simulink model "rfsoc4x2_ospfb_128"  (R2021a)
(part 12 of 339)

  pol1_in1_tap11/2(sync_out) -> pol1_in1_tap12/2(sync)
  pol1_in1_tap11/1(dout) -> pol1_in1_tap12/1(din)
  pol1_in1_first_tap5/6(pot_en_out) -> pol1_in1_tap11/5(pot_en_in)
  [addr] -> pol1_in1_first_tap5/4(addr_in)
  pol1_in1_tap12/4(taps_out) -> delay32/1
  delay29/1 -> adder_1_6/1(sync)
  delay26/1 -> adder_1_5/2(din1)
  pol1_in1_last_tap4/1(tap_out) -> adder_1_5/5(din4)
  pol1_in1_first_tap4/1(dout) -> pol1_in1_tap9/1(din)
  pol1_in2_coeffs3/2(sync_out) -> pol1_in1_first_tap4/2(sync)
  pol1_in1_tap9/3(coeff_out) -> pol1_in1_tap10/3(coeff)
  pol1_in1_first_tap4/2(sync_out) -> pol1_in1_tap9/2(sync)
  pol1_in1_tap10/1(dout) -> pol1_in1_last_tap4/1(din)
  pol1_in1_tap9/5(add_out) -> pol1_in1_tap10/4(addr_in)
  pol1_in1_tap9/6(pot_en_out) -> pol1_in1_tap10/5(pot_en_in)
  pol1_in1_tap10/2(sync_out) -> pol1_in1_last_tap4/2(sync)
  pol1_in1_tap10/3(coeff_out) -> pol1_in1_last_tap4/3(coeff)
  pol1_in2_coeffs3/3(coeff) -> pol1_in1_first_tap4/3(coeffs)
  pol1_in1_last_tap4/2(sync_out) -> delay25/1
  pol1_in1_first_tap4/3(coeff_out) -> pol1_in1_tap9/3(coeff)
  delay27/1 -> adder_1_5/3(din2)
  [tap_write_en] -> pol1_in1_first_tap4/5(pot_en_in)
  pol1_in2_coeffs3/1(dout) -> pol1_in1_first_tap4/1(din)
  delay28/1 -> adder_1_5/4(din3)
  pol1_in1_tap9/4(taps_out) -> delay27/1
  pol1_in1_first_tap4/4(taps_out) -> delay26/1
  pol1_in1_first_tap4/5(add_out) -> pol1_in1_tap9/4(addr_in)
  pol1_in1_tap9/2(sync_out) -> pol1_in1_tap10/2(sync)
  pol1_in1_tap9/1(dout) -> pol1_in1_tap10/1(din)
  pol1_in1_first_tap4/6(pot_en_out) -> pol1_in1_tap9/5(pot_en_in)
  [addr] -> pol1_in1_first_tap4/4(addr_in)
  pol1_in1_tap10/4(taps_out) -> delay28/1
  delay25/1 -> adder_1_5/1(sync)
  delay22/1 -> adder_1_4/2(din1)
  pol1_in1_last_tap3/1(tap_out) -> adder_1_4/5(din4)
  pol1_in1_first_tap3/1(dout) -> pol1_in1_tap7/1(din)
  pol1_in2_coeffs2/2(sync_out) -> pol1_in1_first_tap3/2(sync)
  pol1_in1_tap7/3(coeff_out) -> pol1_in1_tap8/3(coeff)
  pol1_in1_first_tap3/2(sync_out) -> pol1_in1_tap7/2(sync)
  pol1_in1_tap8/1(dout) -> pol1_in1_last_tap3/1(din)
  pol1_in1_tap7/5(add_out) -> pol1_in1_tap8/4(addr_in)
  pol1_in1_tap7/6(pot_en_out) -> pol1_in1_tap8/5(pot_en_in)
  pol1_in1_tap8/2(sync_out) -> pol1_in1_last_tap3/2(sync)
  pol1_in1_tap8/3(coeff_out) -> pol1_in1_last_tap3/3(coeff)
  pol1_in2_coeffs2/3(coeff) -> pol1_in1_first_tap3/3(coeffs)
  pol1_in1_last_tap3/2(sync_out) -> delay21/1
  pol1_in1_first_tap3/3(coeff_out) -> pol1_in1_tap7/3(coeff)
  delay23/1 -> adder_1_4/3(din2)
  [tap_write_en] -> pol1_in1_first_tap3/5(pot_en_in)
  pol1_in2_coeffs2/1(dout) -> pol1_in1_first_tap3/1(din)
  delay24/1 -> adder_1_4/4(din3)
  pol1_in1_tap7/4(taps_out) -> delay23/1
  pol1_in1_first_tap3/4(taps_out) -> delay22/1
  pol1_in1_first_tap3/5(add_out) -> pol1_in1_tap7/4(addr_in)
  pol1_in1_tap7/2(sync_out) -> pol1_in1_tap8/2(sync)
  pol1_in1_tap7/1(dout) -> pol1_in1_tap8/1(din)
  pol1_in1_first_tap3/6(pot_en_out) -> pol1_in1_tap7/5(pot_en_in)
  [addr] -> pol1_in1_first_tap3/4(addr_in)
  pol1_in1_tap8/4(taps_out) -> delay24/1
  delay21/1 -> adder_1_4/1(sync)
  delay18/1 -> adder_1_3/2(din1)
  pol1_in1_last_tap2/1(tap_out) -> adder_1_3/5(din4)
  pol1_in1_first_tap2/1(dout) -> pol1_in1_tap5/1(din)
  pol1_in2_coeffs1/2(sync_out) -> pol1_in1_first_tap2/2(sync)
  pol1_in1_tap5/3(coeff_out) -> pol1_in1_tap6/3(coeff)
  pol1_in1_first_tap2/2(sync_out) -> pol1_in1_tap5/2(sync)
  pol1_in1_tap6/1(dout) -> pol1_in1_last_tap2/1(din)
  pol1_in1_tap5/5(add_out) -> pol1_in1_tap6/4(addr_in)
  pol1_in1_tap5/6(pot_en_out) -> pol1_in1_tap6/5(pot_en_in)
  pol1_in1_tap6/2(sync_out) -> pol1_in1_last_tap2/2(sync)
  pol1_in1_tap6/3(coeff_out) -> pol1_in1_last_tap2/3(coeff)
  pol1_in2_coeffs1/3(coeff) -> pol1_in1_first_tap2/3(coeffs)
  pol1_in1_last_tap2/2(sync_out) -> delay17/1
  pol1_in1_first_tap2/3(coeff_out) -> pol1_in1_tap5/3(coeff)
  delay19/1 -> adder_1_3/3(din2)
  [tap_write_en] -> pol1_in1_first_tap2/5(pot_en_in)
  pol1_in2_coeffs1/1(dout) -> pol1_in1_first_tap2/1(din)
  delay20/1 -> adder_1_3/4(din3)
  pol1_in1_tap5/4(taps_out) -> delay19/1
  pol1_in1_first_tap2/4(taps_out) -> delay18/1
  pol1_in1_first_tap2/5(add_out) -> pol1_in1_tap5/4(addr_in)
  pol1_in1_tap5/2(sync_out) -> pol1_in1_tap6/2(sync)
  pol1_in1_tap5/1(dout) -> pol1_in1_tap6/1(din)
  pol1_in1_first_tap2/6(pot_en_out) -> pol1_in1_tap5/5(pot_en_in)
  [addr] -> pol1_in1_first_tap2/4(addr_in)
  pol1_in1_tap6/4(taps_out) -> delay20/1
  delay17/1 -> adder_1_3/1(sync)
  pol1_in1_last_tap1/1(tap_out) -> adder_1_2/5(din4)
  delay10/1 -> adder_1_2/1(sync)
  [tap_write_en] -> pol1_in1_first_tap1/5(pot_en_in)
  pol1_in1_tap4/4(taps_out) -> delay13/1
  pol1_in1_first_tap1/1(dout) -> pol1_in1_tap1/1(din)
  pol1_in1_tap1/4(taps_out) -> delay12/1
  pol1_in2_coeffs/1(dout) -> pol1_in1_first_tap1/1(din)
  pol1_in1_first_tap1/2(sync_out) -> pol1_in1_tap1/2(sync)
  delay13/1 -> adder_1_2/4(din3)
  pol1_in1_tap1/2(sync_out) -> pol1_in1_tap4/2(sync)
  pol1_in1_tap1/3(coeff_out) -> pol1_in1_tap4/3(coeff)
  pol1_in1_tap4/2(sync_out) -> pol1_in1_last_tap1/2(sync)
  pol1_in2_coeffs/3(coeff) -> pol1_in1_first_tap1/3(coeffs)
  pol1_in1_tap4/1(dout) -> pol1_in1_last_tap1/1(din)
  pol1_in1_first_tap1/5(add_out) -> pol1_in1_tap1/4(addr_in)
  pol1_in1_tap1/5(add_out) -> pol1_in1_tap4/4(addr_in)
  pol1_in1_tap1/1(dout) -> pol1_in1_tap4/1(din)
  pol1_in1_tap1/6(pot_en_out) -> pol1_in1_tap4/5(pot_en_in)
  delay12/1 -> adder_1_2/3(din2)
  pol1_in1_first_tap1/6(pot_en_out) -> pol1_in1_tap1/5(pot_en_in)
  pol1_in1_first_tap1/4(taps_out) -> delay11/1
  pol1_in2_coeffs/2(sync_out) -> pol1_in1_first_tap1/2(sync)
  pol1_in1_tap4/3(coeff_out) -> pol1_in1_last_tap1/3(coeff)
  delay11/1 -> adder_1_2/2(din1)
  pol1_in1_first_tap1/3(coeff_out) -> pol1_in1_tap1/3(coeff)
  [addr] -> pol1_in1_first_tap1/4(addr_in)
  pol1_in1_last_tap1/2(sync_out) -> delay10/1
  Gateway Out6/1 -> scope4/3
  Gateway Out5/1 -> scope4/2
  Gateway Out4/1 -> scope4/4
  Gateway Out7/1 -> scope4/1
  delay7/1 -> Gateway Out7/1, adder_1_1/2(din1)
  delay8/1 -> Gateway Out5/1, adder_1_1/3(din2)
  delay9/1 -> adder_1_1/4(din3), Gateway Out6/1
  Gateway Out3/1 -> scope3/1
  Gateway Out2/1 -> scope2/1
  delay6/1 -> Gateway Out1/1, adder_1_1/1(sync)
  pol1_in1_last_tap/2(sync_out) -> delay6/1
  Gateway Out1/1 -> scope1/1
  delay5/1 -> Gateway Out266/1
  delay4/1 -> Gateway Out265/1
  delay3/1 -> Gateway Out267/1
  pol1_in1_coeffs/1(dout) -> pol1_in1_first_tap/1(din), delay3/1
  Gateway Out267/1 -> scope93/1
  Gateway Out264/1 -> scope93/4
  Gateway Out265/1 -> scope93/2
  Gateway Out266/1 -> scope93/3
  pol1_in1_tap2/6(pot_en_out) -> pol1_in1_tap3/5(pot_en_in)
  pol1_in1_tap2/5(add_out) -> pol1_in1_tap3/4(addr_in)
  pol1_in1_first_tap/6(pot_en_out) -> pol1_in1_tap2/5(pot_en_in)
  pol1_in1_first_tap/5(add_out) -> pol1_in1_tap2/4(addr_in)
  [tap_write_en] -> pol1_in1_first_tap/5(pot_en_in)
  [addr] -> pol1_in1_first_tap/4(addr_in)
  delay2/1 -> Counter38/1, Counter36/1
  Counter38/1 -> Delay26/1, Slice20/1
  Constant61/1 -> Relational11/2
  Slice20/1 -> edge_detect8/1(in)
  Constant63/1 -> Relational12/2
  Gateway Out251/1 -> scope86/1
  edge_detect8/1(out) -> Logical11/2
  Logical11/1 -> Counter36/2
  Gateway Out250/1 -> scope89/1
  AddSub11/1 -> Gateway Out250/1, Relational11/1, Mux3/2, AddSub12/1
  Inverter/1 -> Gateway Out255/1, [tap_write_en]
  Gateway Out252/1 -> scope88/1
  AddSub12/1 -> Mux3/3
  Gateway Out255/1 -> scope90/1
  Mux3/1 -> Gateway Out251/1, [addr]
  Delay27/1 -> Logical11/1
  Relational12/1 -> Inverter/1
  Counter36/1 -> Gateway Out253/1, AddSub11/2
  Constant62/1 -> AddSub12/2
  Gateway Out253/1 -> scope85/1
  Relational11/1 -> Mux3/1
  Delay26/1 -> Gateway Out252/1, AddSub11/1, Relational12/1
  en_ctrl/1 -> Delay27/1
  pol1_in1_tap3/4(taps_out) -> delay9/1
  pol1_in1_tap3/3(coeff_out) -> pol1_in1_last_tap/3(coeff)
  pol1_in1_tap3/2(sync_out) -> pol1_in1_last_tap/2(sync)
  pol1_in1_tap3/1(dout) -> Gateway Out264/1, pol1_in1_last_tap/1(din)
  pol1_in1_last_tap/1(tap_out) -> adder_1_1/5(din4), Gateway Out4/1
  pol1_in1_tap2/4(taps_out) -> delay8/1
  pol1_in1_tap2/3(coeff_out) -> pol1_in1_tap3/3(coeff)
  pol1_in1_tap2/2(sync_out) -> pol1_in1_tap3/2(sync)
  pol1_in1_tap2/1(dout) -> pol1_in1_tap3/1(din), delay5/1
  pol1_in1_first_tap/4(taps_out) -> delay7/1
  pol1_in1_first_tap/3(coeff_out) -> pol1_in1_tap2/3(coeff)
  pol1_in1_first_tap/2(sync_out) -> pol1_in1_tap2/2(sync)
  pol1_in1_first_tap/1(dout) -> pol1_in1_tap2/1(din), delay4/1
  convert_1_16/1 -> pol1_out16/1
  scale_1_16/1 -> convert_1_16/1
  adder_1_16/2(dout) -> scale_1_16/1
  convert_1_15/1 -> pol1_out15/1
  scale_1_15/1 -> convert_1_15/1
  adder_1_15/2(dout) -> scale_1_15/1
  convert_1_14/1 -> pol1_out14/1
  scale_1_14/1 -> convert_1_14/1
  adder_1_14/2(dout) -> scale_1_14/1
  convert_1_13/1 -> pol1_out13/1
  scale_1_13/1 -> convert_1_13/1
  adder_1_13/2(dout) -> scale_1_13/1
  convert_1_12/1 -> pol1_out12/1
  scale_1_12/1 -> convert_1_12/1
  adder_1_12/2(dout) -> scale_1_12/1
  convert_1_11/1 -> pol1_out11/1
  scale_1_11/1 -> convert_1_11/1
  adder_1_11/2(dout) -> scale_1_11/1
  convert_1_10/1 -> pol1_out10/1
  scale_1_10/1 -> convert_1_10/1
  adder_1_10/2(dout) -> scale_1_10/1
  convert_1_9/1 -> pol1_out9/1
  scale_1_9/1 -> convert_1_9/1
  adder_1_9/2(dout) -> scale_1_9/1
  convert_1_8/1 -> pol1_out8/1
  scale_1_8/1 -> convert_1_8/1
  adder_1_8/2(dout) -> scale_1_8/1
  convert_1_7/1 -> pol1_out7/1
  scale_1_7/1 -> convert_1_7/1
  adder_1_7/2(dout) -> scale_1_7/1
  convert_1_6/1 -> pol1_out6/1
  scale_1_6/1 -> convert_1_6/1
  adder_1_6/2(dout) -> scale_1_6/1
  convert_1_5/1 -> pol1_out5/1
  scale_1_5/1 -> convert_1_5/1
  adder_1_5/2(dout) -> scale_1_5/1
  convert_1_4/1 -> pol1_out4/1
  scale_1_4/1 -> convert_1_4/1
  adder_1_4/2(dout) -> scale_1_4/1
  convert_1_3/1 -> pol1_out3/1
  scale_1_3/1 -> convert_1_3/1
  adder_1_3/2(dout) -> scale_1_3/1
  convert_1_2/1 -> pol1_out2/1
  scale_1_2/1 -> convert_1_2/1
  adder_1_2/2(dout) -> scale_1_2/1
  convert_1_1/1 -> pol1_out1/1, Gateway Out3/1
  scale_1_1/1 -> convert_1_1/1
  adder_1_1/2(dout) -> scale_1_1/1
  delay1/1 -> sync_out/1, Gateway Out2/1
  adder_1_1/1(sync_out) -> delay1/1
  pol1_in16/1 -> pol1_in2_coeffs14/1(din)
  pol1_in15/1 -> pol1_in2_coeffs13/1(din)
  pol1_in14/1 -> pol1_in2_coeffs12/1(din)
  pol1_in13/1 -> pol1_in2_coeffs11/1(din)
  pol1_in12/1 -> pol1_in2_coeffs10/1(din)
  pol1_in11/1 -> pol1_in2_coeffs9/1(din)
  pol1_in10/1 -> pol1_in2_coeffs8/1(din)
  pol1_in9/1 -> pol1_in2_coeffs7/1(din)
  pol1_in8/1 -> pol1_in2_coeffs6/1(din)
  pol1_in7/1 -> pol1_in2_coeffs5/1(din)
  pol1_in6/1 -> pol1_in2_coeffs4/1(din)
  pol1_in5/1 -> pol1_in2_coeffs3/1(din)
  pol1_in4/1 -> pol1_in2_coeffs2/1(din)
  pol1_in3/1 -> pol1_in2_coeffs1/1(din)
  pol1_in2/1 -> pol1_in2_coeffs/1(din)
  pol1_in1_coeffs/3(coeff) -> pol1_in1_first_tap/3(coeffs)
  pol1_in1_coeffs/2(sync_out) -> pol1_in1_first_tap/2(sync)
  sync/1 -> pol1_in2_coeffs10/2(sync), pol1_in2_coeffs11/2(sync), pol1_in2_coeffs12/2(sync), pol1_in2_coeffs14/2(sync), pol1_in2_coeffs13/2(sync), pol1_in2_coeffs9/2(sync), pol1_in2_coeffs8/2(sync), pol1_in2_coeffs7/2(sync), pol1_in2_coeffs6/2(sync), pol1_in2_coeffs5/2(sync), pol1_in2_coeffs4/2(sync), pol1_in2_coeffs3/2(sync), pol1_in2_coeffs2/2(sync), pol1_in2_coeffs1/2(sync), pol1_in2_coeffs/2(sync), pol1_in1_coeffs/2(sync), delay2/1
  pol1_in1/1 -> pol1_in1_coeffs/1(din)
  Gateway Out13/1 -> scope6/2
  Gateway Out14/1 -> scope6/3
  delay73/1 -> Gateway Out15/1
  delay75/1 -> Gateway Out14/1
  Gateway Out15/1 -> scope6/1
  delay74/1 -> Gateway Out13/1
  Gateway Out12/1 -> scope6/4
  Gateway Out19/1 -> scope6/5
  Gateway Out17/1 -> scope6/6
  Gateway Out18/1 -> scope6/7
  Gateway Out16/1 -> scope6/8
  Slice/1 -> Reinterpret/1
  Reinterpret/1 -> Gateway Out19/1
  Slice1/1 -> Reinterpret1/1
  Reinterpret1/1 -> Gateway Out17/1
  Slice2/1 -> Reinterpret2/1
  Reinterpret2/1 -> Gateway Out18/1
  Reinterpret3/1 -> Gateway Out16/1
